simulink model "PID_SIMULINK"  (R2023b)
settings: Solver=VariableStepAuto  StartTime=0.0  StopTime=50  RelTol=1e-3
values from neighbouring files (symbols this model uses):
  D_LONG = -0.469    [PIDComplelto.m]    (also in get_pid_metrics.m)
  k_r = -0.174    [PIDComplelto.m]    (also in get_pid_metrics.m)
  K_roll = -0.106    [PIDComplelto.m]    (also in PID_lat.m = 0.106; get_pid_metrics.m)
  linmodel =     [modelo_lin.mat]
undefined symbols (not defined in the file or in its folder): Den_LONG, Den_ROLL, Den_YAW, Num_LONG, Num_ROLL, Num_YAW
libraries: simulink x4
settings Model: Creator=sslan  LastModifiedBy=sslan

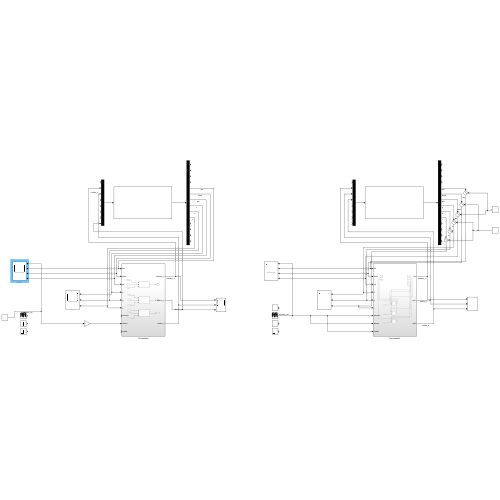
[thumbnail: Simulink's stored preview of the top-level diagram]
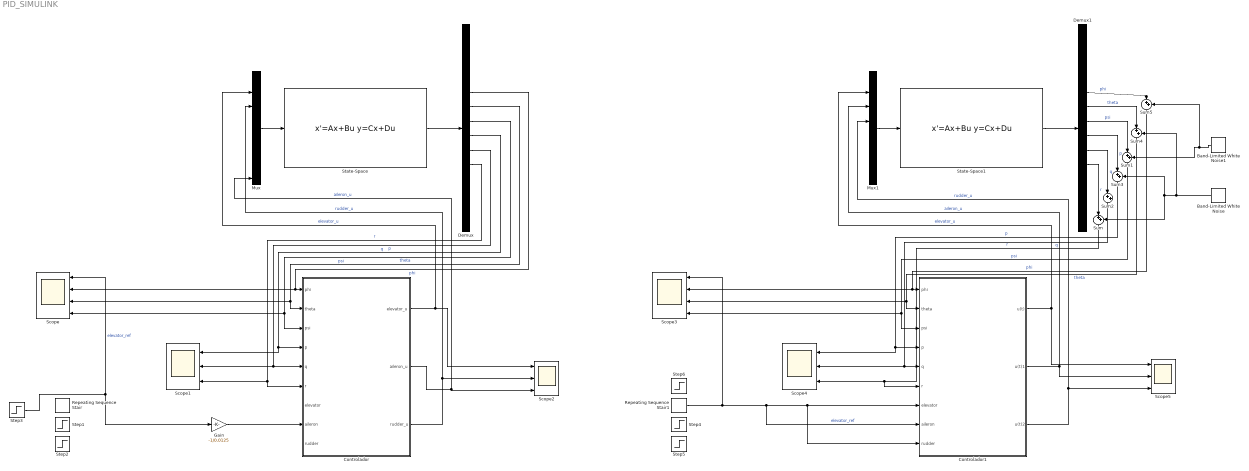
== system PID_SIMULINK ==
  Band-Limited White Noise : simulink/Sources/Band-Limited White Noise  Cov=[0.001]  Ts=0.1  seed=[23341]
  Band-Limited White Noise1 : simulink/Sources/Band-Limited White Noise  Cov=[0.0001]  Ts=0.1  seed=[23341]
  Controlador : Subsystem
  Controlador1 : Subsystem
  Demux : Demux  Outputs=14
  Demux1 : Demux  Outputs=14
  Gain : Gain  Gain=-1/0.0125
  Mux : Mux  Inputs=8
  Mux1 : Mux  Inputs=8
  Repeating Sequence Stair : simulink/Sources/Repeating Sequence Stair  OutValues=[2 2 -2 2 2 -2].'  tsamp=10  OutMin=[]  OutMax=[]  OutDataTypeStr=double  OutputDataTypeScalingMode=double  OutDataType=fixdt(0,8)  ConRadixGroup=Best Precision: Vector-wise  OutScaling=2^-12
  Repeating Sequence Stair1 : simulink/Sources/Repeating Sequence Stair  OutValues=[2 2 -2 2 2 -2].'  tsamp=10  OutMin=[]  OutMax=[]  OutDataTypeStr=double  OutputDataTypeScalingMode=double  OutDataType=fixdt(0,8)  ConRadixGroup=Best Precision: Vector-wise  OutScaling=2^-12
  Scope : Scope  NumInputPorts=4
  Scope{1..2,4..5} (4 alike) : Scope  NumInputPorts=3
  Scope3 : Scope  NumInputPorts=4
  State-Space : StateSpace  A=linmodel.A  B=linmodel.B  C=linmodel.C  D=linmodel.D  InitialCondition=0
  State-Space1 : StateSpace  A=linmodel.A  B=linmodel.B  C=linmodel.C  D=linmodel.D  InitialCondition=0
  Step{1..2,4..5} (4 alike) : Step  After=40  SampleTime=0
  Step3 : Step  Time=15  Before=-40  After=20  SampleTime=0
  Step6 : Step  Before=-40  After=40  SampleTime=0
  Sum{,1..5} (6 alike) : Sum  Inputs=|++
  wires:
  Mux/1 -> State-Space/1
  State-Space/1 -> Demux/1
  Demux/6 -> Controlador/2(theta), Scope/3  "theta"
  Demux/7 -> Controlador/3(psi), Scope/4  "psi"
  Demux/8 -> Scope1/1, Controlador/4(p)  "p"
  Demux/9 -> Controlador/5(q), Scope1/2  "q"
  Demux/10 -> Controlador/6(r), Scope1/3  "r"
  Step3/1 -> Gain/1, Scope/1  "elevator_ref"
  Controlador/1(elevator_u) -> Scope2/1, Mux/2  "elevator_u"
  Controlador/3(rudder_u) -> Mux/3, Scope2/2  "rudder_u"
  Controlador/2(aileron_u) -> Scope2/3, Mux/8  "aileron_u"
  Demux/5 -> Controlador/1(phi), Scope/2  "phi"
  Repeating Sequence Stair1/1 -> Scope3/1, Controlador1/8(aileron), Controlador1/9(rudder), Controlador1/7(elevator)  "elevator_ref"
  Controlador1/2(u(t)1) -> Scope5/2, Mux1/3  "aileron_u"
  Sum/1 -> Controlador1/6(r), Scope4/3  "r"
  Sum5/1 -> Controlador1/1(phi), Scope3/2  "phi"
  Controlador1/3(u(t)2) -> Scope5/3, Mux1/4  "rudder_u"
  Mux1/1 -> State-Space1/1
  Controlador1/1(u(t)) -> Scope5/1, Mux1/2  "elevator_u"
  State-Space1/1 -> Demux1/1
  Sum2/1 -> Scope4/2, Controlador1/5(q)  "q"
  Sum4/1 -> Controlador1/2(theta), Scope3/3  "theta"
  Sum1/1 -> Controlador1/3(psi), Scope3/4  "psi"
  Sum3/1 -> Scope4/1, Controlador1/4(p)  "p"
  Demux1/10 -> Sum/1  "r"
  Band-Limited White Noise/1 -> Sum4/2, Sum3/2, Sum/2
  Demux1/9 -> Sum2/1  "q"
  Demux1/8 -> Sum3/1  "p"
  Demux1/7 -> Sum1/1  "psi"
  Demux1/6 -> Sum4/1  "theta"
  Demux1/5 -> Sum5/1  "phi"
  Band-Limited White Noise1/1 -> Sum5/2, Sum1/2
  Gain/1 -> Controlador/8(aileron)

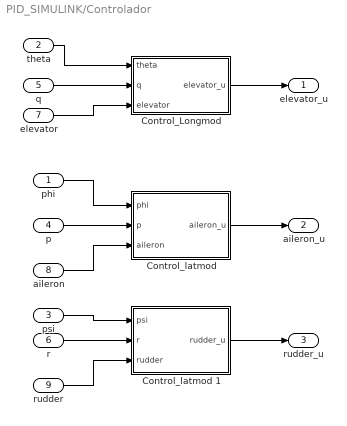
== system PID_SIMULINK/Controlador ==
  phi : Inport
  theta : Inport  Port=2
  psi : Inport  Port=3
  p : Inport  Port=4
  q : Inport  Port=5
  r : Inport  Port=6
  elevator : Inport  Port=7
  aileron : Inport  Port=8
  rudder : Inport  Port=9
  Control_Longmod : Subsystem
  "Control_latmod " : Subsystem
  Control_latmod 1 : Subsystem
  elevator_u : Outport
  aileron_u : Outport  Port=2
  rudder_u : Outport  Port=3
  wires:
  rudder/1 -> Control_latmod 1/3(rudder)
  aileron/1 -> "Control_latmod "/3(aileron)
  r/1 -> Control_latmod 1/2(r)
  p/1 -> "Control_latmod "/2(p)
  elevator/1 -> Control_Longmod/3(elevator)
  phi/1 -> "Control_latmod "/1(phi)
  theta/1 -> Control_Longmod/1(theta)
  q/1 -> Control_Longmod/2(q)
  Control_Longmod/1(elevator_u) -> elevator_u/1
  psi/1 -> Control_latmod 1/1(psi)
  "Control_latmod "/1(aileron_u) -> aileron_u/1
  Control_latmod 1/1(rudder_u) -> rudder_u/1

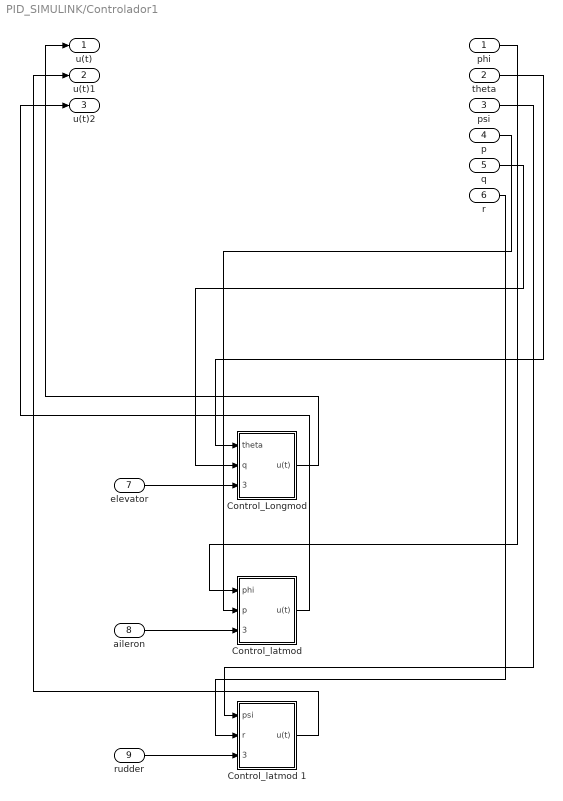
== system PID_SIMULINK/Controlador1 ==
  phi : Inport
  theta : Inport  Port=2
  psi : Inport  Port=3
  p : Inport  Port=4
  q : Inport  Port=5
  r : Inport  Port=6
  elevator : Inport  Port=7
  aileron : Inport  Port=8
  rudder : Inport  Port=9
  Control_Longmod : Subsystem
  "Control_latmod " : Subsystem
  Control_latmod 1 : Subsystem
  u(t) : Outport
  u(t)1 : Outport  Port=2
  u(t)2 : Outport  Port=3
  wires:
  rudder/1 -> Control_latmod 1/3(rudder)
  aileron/1 -> "Control_latmod "/3(aileron)
  r/1 -> Control_latmod 1/2(r)
  p/1 -> "Control_latmod "/2(p)
  elevator/1 -> Control_Longmod/3(elevator)
  "Control_latmod "/1(u(t)) -> u(t)2/1
  phi/1 -> "Control_latmod "/1(phi)
  Control_latmod 1/1(u(t)) -> u(t)1/1
  theta/1 -> Control_Longmod/1(theta)
  q/1 -> Control_Longmod/2(q)
  Control_Longmod/1(u(t)) -> u(t)/1
  psi/1 -> Control_latmod 1/1(psi)

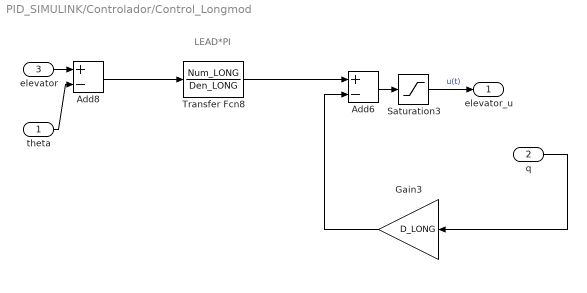
== system PID_SIMULINK/Controlador/Control_Longmod ==
  note: LEAD*PI
  theta : Inport
  q : Inport  Port=2
  elevator : Inport  Port=3
  Add6 : Sum  Inputs=+-
  Add8 : Sum  Inputs=+-
  Gain3 : Gain  Gain=D_LONG
  Saturation3 : Saturate  UpperLimit=30  LowerLimit=-30
  Transfer Fcn8 : TransferFcn  Numerator=Num_LONG  Denominator=Den_LONG
  elevator_u : Outport
  wires:
  Transfer Fcn8/1 -> Add6/1
  Gain3/1 -> Add6/2
  Saturation3/1 -> elevator_u/1  "u(t)"
  Add6/1 -> Saturation3/1
  Add8/1 -> Transfer Fcn8/1
  q/1 -> Gain3/1
  elevator/1 -> Add8/1
  theta/1 -> Add8/2

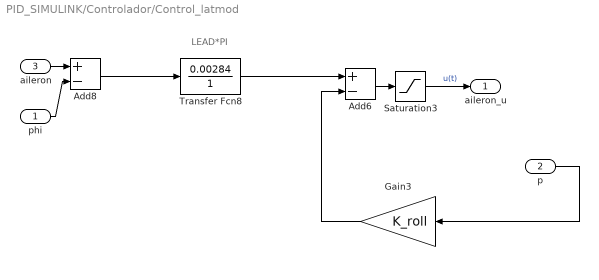
== system PID_SIMULINK/Controlador/Control_latmod  ==
  note: LEAD*PI
  phi : Inport
  p : Inport  Port=2
  aileron : Inport  Port=3
  Add6 : Sum  Inputs=+-
  Add8 : Sum  Inputs=+-
  Gain3 : Gain  Gain=K_roll
  Saturation3 : Saturate  UpperLimit=30  LowerLimit=-30
  Transfer Fcn8 : TransferFcn  Numerator=0.00284  Denominator=1
  aileron_u : Outport
  wires:
  Transfer Fcn8/1 -> Add6/1
  Gain3/1 -> Add6/2
  Saturation3/1 -> aileron_u/1  "u(t)"
  Add6/1 -> Saturation3/1
  Add8/1 -> Transfer Fcn8/1
  p/1 -> Gain3/1
  aileron/1 -> Add8/1
  phi/1 -> Add8/2

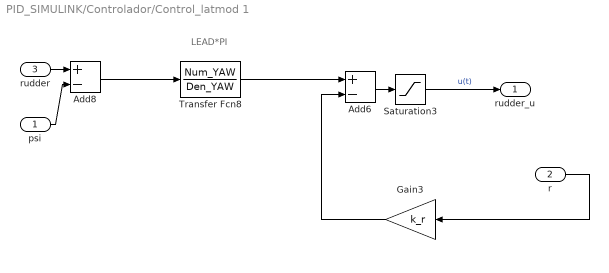
== system PID_SIMULINK/Controlador/Control_latmod 1 ==
  note: LEAD*PI
  psi : Inport
  r : Inport  Port=2
  rudder : Inport  Port=3
  Add6 : Sum  Inputs=+-
  Add8 : Sum  Inputs=+-
  Gain3 : Gain  Gain=k_r
  Saturation3 : Saturate  UpperLimit=30  LowerLimit=-30
  Transfer Fcn8 : TransferFcn  Numerator=Num_YAW  Denominator=Den_YAW
  rudder_u : Outport
  wires:
  Transfer Fcn8/1 -> Add6/1
  Gain3/1 -> Add6/2
  Saturation3/1 -> rudder_u/1  "u(t)"
  Add6/1 -> Saturation3/1
  Add8/1 -> Transfer Fcn8/1
  r/1 -> Gain3/1
  rudder/1 -> Add8/1
  psi/1 -> Add8/2

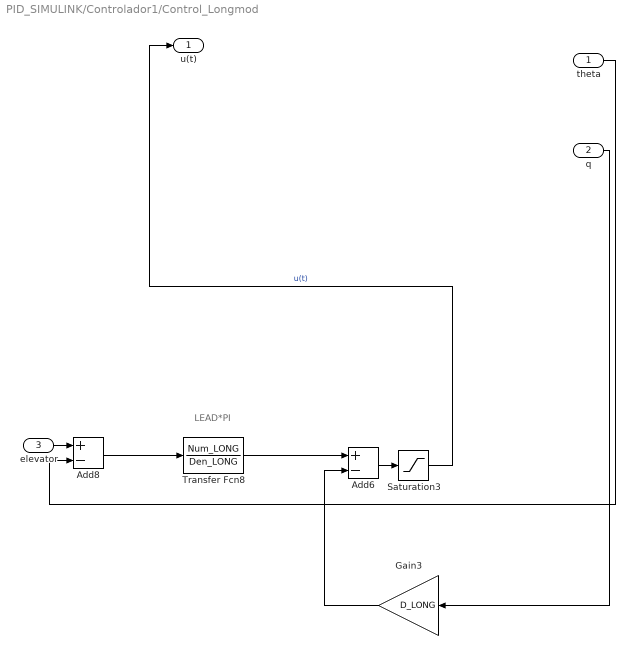
== system PID_SIMULINK/Controlador1/Control_Longmod ==
  note: LEAD*PI
  theta : Inport
  q : Inport  Port=2
  elevator : Inport  Port=3
  Add6 : Sum  Inputs=+-
  Add8 : Sum  Inputs=+-
  Gain3 : Gain  Gain=D_LONG
  Saturation3 : Saturate  UpperLimit=30  LowerLimit=-30
  Transfer Fcn8 : TransferFcn  Numerator=Num_LONG  Denominator=Den_LONG
  u(t) : Outport
  wires:
  Transfer Fcn8/1 -> Add6/1
  Gain3/1 -> Add6/2
  Saturation3/1 -> u(t)/1  "u(t)"
  Add6/1 -> Saturation3/1
  Add8/1 -> Transfer Fcn8/1
  q/1 -> Gain3/1
  elevator/1 -> Add8/1
  theta/1 -> Add8/2

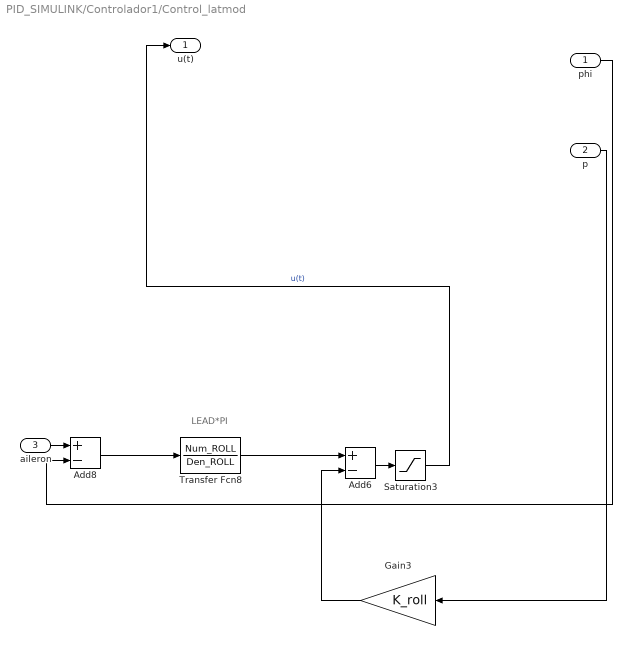
== system PID_SIMULINK/Controlador1/Control_latmod  ==
  note: LEAD*PI
  phi : Inport
  p : Inport  Port=2
  aileron : Inport  Port=3
  Add6 : Sum  Inputs=+-
  Add8 : Sum  Inputs=+-
  Gain3 : Gain  Gain=K_roll
  Saturation3 : Saturate  UpperLimit=30  LowerLimit=-30
  Transfer Fcn8 : TransferFcn  Numerator=Num_ROLL  Denominator=Den_ROLL
  u(t) : Outport
  wires:
  Transfer Fcn8/1 -> Add6/1
  Gain3/1 -> Add6/2
  Saturation3/1 -> u(t)/1  "u(t)"
  Add6/1 -> Saturation3/1
  Add8/1 -> Transfer Fcn8/1
  p/1 -> Gain3/1
  aileron/1 -> Add8/1
  phi/1 -> Add8/2

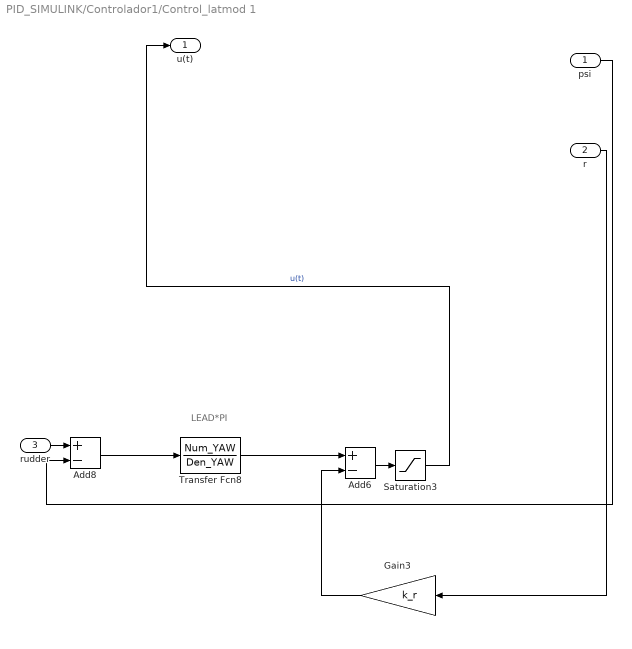
== system PID_SIMULINK/Controlador1/Control_latmod 1 ==
  note: LEAD*PI
  psi : Inport
  r : Inport  Port=2
  rudder : Inport  Port=3
  Add6 : Sum  Inputs=+-
  Add8 : Sum  Inputs=+-
  Gain3 : Gain  Gain=k_r
  Saturation3 : Saturate  UpperLimit=30  LowerLimit=-30
  Transfer Fcn8 : TransferFcn  Numerator=Num_YAW  Denominator=Den_YAW
  u(t) : Outport
  wires:
  Transfer Fcn8/1 -> Add6/1
  Gain3/1 -> Add6/2
  Saturation3/1 -> u(t)/1  "u(t)"
  Add6/1 -> Saturation3/1
  Add8/1 -> Transfer Fcn8/1
  r/1 -> Gain3/1
  rudder/1 -> Add8/1
  psi/1 -> Add8/2
